simulink model "day11p2"  (R2026a)
settings: Solver=FixedStepAuto  StopTime=inf
InitFcn:
  | QueueLen = 200;
  | 
  | %{
  | fxp: udl vii hgb qmy
  | ixc: cje lra jhu
  | sgn: apv vbc
  | wua: knq
  | fnr: csd awl vvj fyx cvi xhb mvn guw wid vbp uvk krt oil izj zlh gwv
  | krt: grp cml vxt
  | hwj: laq jlg
  | rus: out
  | oag: wrc gpp
  | uos: zqg aiu gdx
  | xpu: qpb zqg gdx aiu
  | mdb: fnr mwu ozd
  | yrt: jlg ifs laq
  | eao: txi jmk xee sta knq
  | qcj: ivn mwb nrx lgx
  | wks: fyy lyd
  | xso: rqn flj fak
  | ucp: wpn mpy
  | zcf: knq sta xee jmk
  | sdr: vfy gsc wfb
  | ggn: brb ylm kdl rnk
  | tky: wcx ytk hbp xjh dne
  | kzl: sft sof utn
  | epc: uhn cqf xwv
  | srh: shh mei
  | uqe: sft
  | htw: hmf aia wsm
  | wid: qwo
  | daz: yvs
  | bdl: ipm kkp
  | xay: mpi
  | bsb: epc jpb cqs ixc cur ril ybr
  | mwb: out
  | cxr: yvs
  | ruf: jax uvl ctm
  | vtp: rbo
  | tqs: kdl pje ylm brb
  | thb: out
  | ljy: ael tqw
  | tkl: ssx yds
  | ozd: itv csd vvj fyx awl xhb mvn guw vbp hzn yft mfv izj oil uvk cui krt myo fqn gwv zlh
  | uhn: lzx dac iqf
  | zad: wvh tmc ece
  | qlf: gce sgn fni
  | kcf: dka pvw uzw
  | uat: bda mkd
  | aai: gtk gkf cuk qcj
  | mfv: cml
  | qlv: wdr sbi ihm nww jkx bud qxb
  | paz: kbq osk
  | rys: iwh
  | gdx: out
  | hco: cuk gkf
  | gte: wks fft
  | zrw: iur mei shh
  | izj: elj wrh vnz uss
  | lur: jpb zib zwl uzn epc nta cur cqs ybr tkl sle
  | ... (+518 lines)
undefined symbols (not defined in the file): DiscIntNeverNeededParam
libraries: simulink x12
(part 4 of 4)

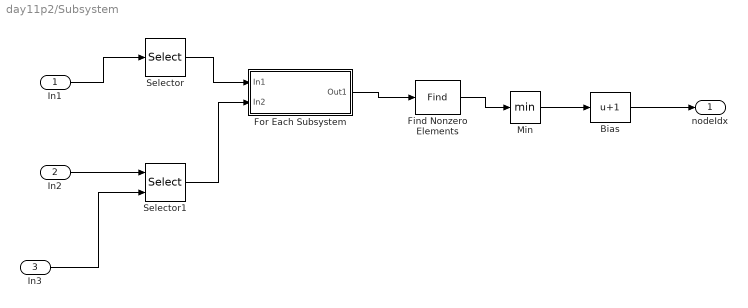
== system day11p2/Subsystem ==
  In1 : Inport
  In2 : Inport  Port=2
  In3 : Inport  Port=3
  Bias : Bias  Bias=1  SaturateOnIntegerOverflow=off
  Find Nonzero Elements : Find  NumberOfInputDimensions=3  IndexMode=Zero-based
  For Each Subsystem : Subsystem  TreatAsAtomicUnit=on
  Min : MinMax
  Selector : Selector  NumberOfDimensions=2  InputPortWidth=3  IndexOptions=Select all,Index vector (dialog)  Indices=[1 3],[1 2 3]  OutputSizes=1,1  RuntimeRangeChecks=on
  Selector1 : Selector  NumberOfDimensions=2  InputPortWidth=3  IndexOptions=Index vector (port),Index vector (dialog)  Indices=1,[1 2 3]  OutputSizes=1,1  RuntimeRangeChecks=on
  nodeIdx : Outport
  wires:
  In1/1 -> Selector/1
  In2/1 -> Selector1/1
  Selector/1 -> For Each Subsystem/1(In1)
  Selector1/1 -> For Each Subsystem/2(In2)
  For Each Subsystem/1(Out1) -> Find Nonzero Elements/1
  Find Nonzero Elements/1 -> Min/1
  Min/1 -> Bias/1
  Bias/1 -> nodeIdx/1
  In3/1 -> Selector1/2

== system day11p2/Subsystem1 ==
  In1 : Inport
  In2 : Inport  Port=2
  Assignment : Assignment  NumberOfDimensions=2  DiagnosticForDimensions=Warning  IndexOptions=Index vector (port),Index vector (dialog)  Indices=1,[1:5]  OutputSizes=1,1  RuntimeRangeChecks=on
  Bias : Bias  Bias=-1  SaturateOnIntegerOverflow=off
  Constant : Constant  Value=[0 0 0 0 0]  VectorParams1D=off
  queue : Outport
  queueLen : Outport  Port=2
  wires:
  In2/1 -> Bias/1, Assignment/3
  Bias/1 -> queueLen/1
  In1/1 -> Assignment/1
  Constant/1 -> Assignment/2
  Assignment/1 -> queue/1

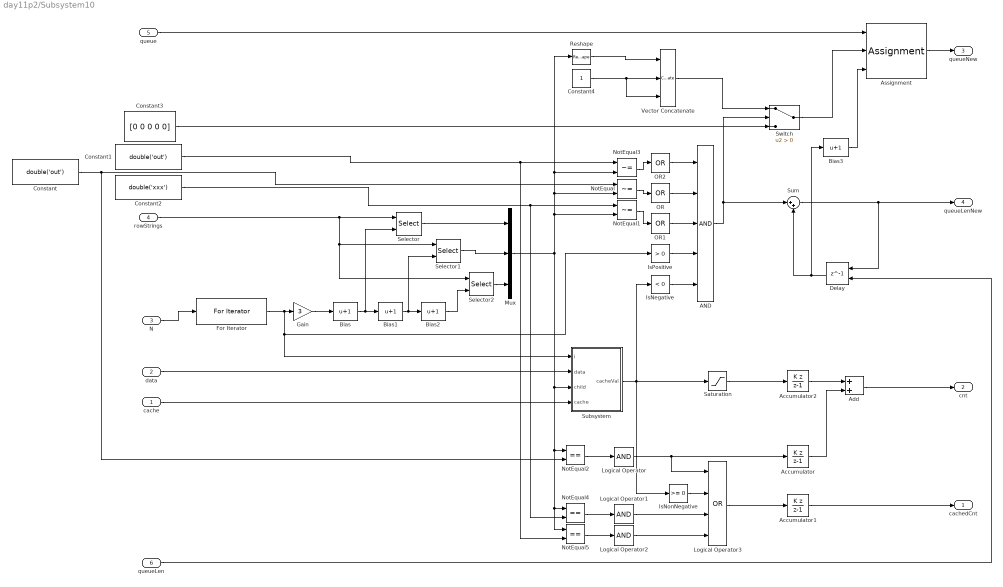
== system day11p2/Subsystem10 ==
  cache : Inport
  data : Inport  Port=2
  N : Inport  Port=3
  rowStrings : Inport  Port=4
  queue : Inport  Port=5
  queueLen : Inport  Port=6
  AND : Logic  Inputs=5  IconShape=distinctive  AllPortsSameDT=off  OutDataTypeStr=boolean
  Accumulator : DiscreteIntegrator  IntegratorMethod=Accumulation: Backward Euler  SampleTime=-1  OutDataTypeStr=double  ICPrevOutput=DiscIntNeverNeededParam  ICPrevScaledInput=DiscIntNeverNeededParam
  Accumulator1 : DiscreteIntegrator  IntegratorMethod=Accumulation: Backward Euler  SampleTime=-1  OutDataTypeStr=double  ICPrevOutput=DiscIntNeverNeededParam  ICPrevScaledInput=DiscIntNeverNeededParam
  Accumulator2 : DiscreteIntegrator  IntegratorMethod=Accumulation: Backward Euler  SampleTime=-1  OutDataTypeStr=double  ICPrevOutput=DiscIntNeverNeededParam  ICPrevScaledInput=DiscIntNeverNeededParam
  Add : Sum
  Assignment : Assignment  NumberOfDimensions=2  DiagnosticForDimensions=Warning  IndexOptions=Index vector (port),Index vector (dialog)  Indices=1,[1 2 3 4 5]  OutputSizes=1,1  RuntimeRangeChecks=on
  Bias{,1..3} (4 alike) : Bias  Bias=1  SaturateOnIntegerOverflow=off
  Constant : Constant  Value=double('out')
  Constant1 : Constant  Value=double('out')
  Constant2 : Constant  Value=double('xxx')
  Constant3 : Constant  Value=[0 0 0 0 0]  VectorParams1D=off
  Constant4 : Constant
  Delay : Delay  DelayLength=1  InitialConditionSource=Input port
      settings: InputPortMap=u0,p4
  For Iterator : ForIterator  ResetStates=reset  IterationSource=external  IndexMode=Zero-based  IterationVariableDataType=double
  Gain : Gain  Gain=3
  IsNegative : simulink/Logic and Bit Operations/Compare To Zero  relop=<  OutDataTypeStr=boolean
      settings: LibrarySourceBlock=|
      | simulink/Quick Insert/Logic and Bit
      | Operations/IsNegative
  IsNonNegative : simulink/Logic and Bit Operations/Compare To Zero  relop=>=  OutDataTypeStr=boolean
      settings: LibrarySourceBlock=|
      | simulink/Quick Insert/Logic and Bit
      | Operations/IsNonNegative
  IsPositive : simulink/Logic and Bit Operations/Compare To Zero  relop=>  OutDataTypeStr=boolean
      settings: LibrarySourceBlock=|
      | simulink/Quick Insert/Logic and Bit
      | Operations/IsPositive
  Logical Operator : Logic  Inputs=1  AllPortsSameDT=off  OutDataTypeStr=boolean
  Logical Operator1 : Logic  Inputs=1  AllPortsSameDT=off  OutDataTypeStr=boolean
  Logical Operator2 : Logic  Inputs=1  AllPortsSameDT=off  OutDataTypeStr=boolean
  Logical Operator3 : Logic  Operator=OR  Inputs=4  AllPortsSameDT=off  OutDataTypeStr=boolean
  Mux : Mux  Inputs=3
  NotEqual : RelationalOperator  Operator=~=  OutDataTypeStr=boolean  RndMeth=Simplest  InputSameDT=off
  NotEqual1 : RelationalOperator  Operator=~=  OutDataTypeStr=boolean  RndMeth=Simplest  InputSameDT=off
  NotEqual2 : RelationalOperator  Operator===  OutDataTypeStr=boolean  RndMeth=Simplest  InputSameDT=off
  NotEqual3 : RelationalOperator  Operator=~=  OutDataTypeStr=boolean  RndMeth=Simplest  InputSameDT=off
  NotEqual4 : RelationalOperator  Operator===  OutDataTypeStr=boolean  RndMeth=Simplest  InputSameDT=off
  NotEqual5 : RelationalOperator  Operator===  OutDataTypeStr=boolean  RndMeth=Simplest  InputSameDT=off
  OR : Logic  Operator=OR  Inputs=1  IconShape=distinctive  AllPortsSameDT=off  OutDataTypeStr=boolean
  OR1 : Logic  Operator=OR  Inputs=1  IconShape=distinctive  AllPortsSameDT=off  OutDataTypeStr=boolean
  OR2 : Logic  Operator=OR  Inputs=1  IconShape=distinctive  AllPortsSameDT=off  OutDataTypeStr=boolean
  Reshape : Reshape  OutputDimensionality=Row vector (2-D)
  Saturation : Saturate  UpperLimit=1e6  LowerLimit=0
  Selector : Selector  NumberOfDimensions=2  InputPortWidth=3  IndexOptions=Select all,Index vector (port)  Indices=[1 3],1  OutputSizes=1,1  RuntimeRangeChecks=on
  Selector1 : Selector  NumberOfDimensions=2  InputPortWidth=3  IndexOptions=Select all,Index vector (port)  Indices=[1 3],1  OutputSizes=1,1  RuntimeRangeChecks=on
  Selector2 : Selector  NumberOfDimensions=2  InputPortWidth=3  IndexOptions=Select all,Index vector (port)  Indices=[1 3],1  OutputSizes=1,1  RuntimeRangeChecks=on
  Subsystem : Subsystem
  Sum : Sum  Inputs=|++
  Switch : Switch  Criteria=u2 > Threshold  SaturateOnIntegerOverflow=off  InputSameDT=off
  Vector Concatenate : Concatenate  NumInputs=3
  cachedCnt : Outport
  cnt : Outport  Port=2
  queueNew : Outport  Port=3
  queueLenNew : Outport  Port=4
  wires:
  N/1 -> For Iterator/1
  Bias/1 -> Selector/2, Bias1/1
  Bias1/1 -> Selector1/2, Bias2/1
  For Iterator/1 -> Subsystem/1(i), IsPositive/1, Gain/1
  Gain/1 -> Bias/1
  rowStrings/1 -> Selector2/1, Selector1/1, Selector/1
  Bias2/1 -> Selector2/2
  Selector/1 -> Mux/1
  Selector1/1 -> Mux/2
  Selector2/1 -> Mux/3
  NotEqual/1 -> OR/1
  NotEqual1/1 -> OR1/1
  Mux/1 -> Reshape/1, NotEqual3/2, NotEqual/2, NotEqual1/2, NotEqual5/1, NotEqual4/1, NotEqual2/1, Subsystem/3(child)
  OR/1 -> AND/2
  OR1/1 -> AND/3
  IsPositive/1 -> AND/4
  Constant2/1 -> NotEqual4/2, NotEqual1/1
  AND/1 -> Sum/1, Switch/2
  Constant3/1 -> Switch/3
  Delay/1 -> Bias3/1, Sum/2
  Sum/1 -> Delay/1, queueLenNew/1
  queueLen/1 -> Delay/2
  queue/1 -> Assignment/1
  Switch/1 -> Assignment/2
  Bias3/1 -> Assignment/3
  Assignment/1 -> queueNew/1
  NotEqual2/1 -> Logical Operator/1
  Constant/1 -> NotEqual/1, NotEqual2/2
  Logical Operator/1 -> Logical Operator3/1, Accumulator/1
  Reshape/1 -> Vector Concatenate/1
  Vector Concatenate/1 -> Switch/1
  Constant4/1 -> Vector Concatenate/3, Vector Concatenate/2
  NotEqual3/1 -> OR2/1
  OR2/1 -> AND/1
  Constant1/1 -> NotEqual5/2, NotEqual3/1
  IsNegative/1 -> AND/5
  NotEqual4/1 -> Logical Operator1/1
  NotEqual5/1 -> Logical Operator2/1
  Logical Operator2/1 -> Logical Operator3/4
  Logical Operator1/1 -> Logical Operator3/3
  IsNonNegative/1 -> Logical Operator3/2
  Logical Operator3/1 -> Accumulator1/1
  Accumulator1/1 -> cachedCnt/1
  cache/1 -> Subsystem/4(cache)
  data/1 -> Subsystem/2(data)
  Subsystem/1(cacheVal) -> Saturation/1, IsNegative/1, IsNonNegative/1
  Saturation/1 -> Accumulator2/1
  Accumulator2/1 -> Add/1
  Accumulator/1 -> Add/2
  Add/1 -> cnt/1

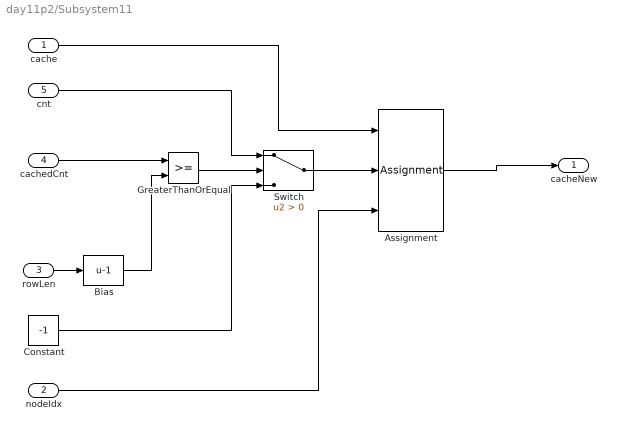
== system day11p2/Subsystem11 ==
  cache : Inport
  nodeIdx : Inport  Port=2
  rowLen : Inport  Port=3
  cachedCnt : Inport  Port=4
  cnt : Inport  Port=5
  Assignment : Assignment  DiagnosticForDimensions=Warning  IndexOptions=Index vector (port)  Indices=1  OutputSizes=1  RuntimeRangeChecks=on
  Bias : Bias  Bias=-1  SaturateOnIntegerOverflow=off
  Constant : Constant  Value=-1
  GreaterThanOrEqual : RelationalOperator  OutDataTypeStr=boolean  RndMeth=Simplest  InputSameDT=off
  Switch : Switch  Criteria=u2 > Threshold  SaturateOnIntegerOverflow=off  InputSameDT=off
  cacheNew : Outport
  wires:
  cachedCnt/1 -> GreaterThanOrEqual/1
  rowLen/1 -> Bias/1
  Bias/1 -> GreaterThanOrEqual/2
  GreaterThanOrEqual/1 -> Switch/2
  cnt/1 -> Switch/1
  Constant/1 -> Switch/3
  Switch/1 -> Assignment/2
  cache/1 -> Assignment/1
  Assignment/1 -> cacheNew/1
  nodeIdx/1 -> Assignment/3

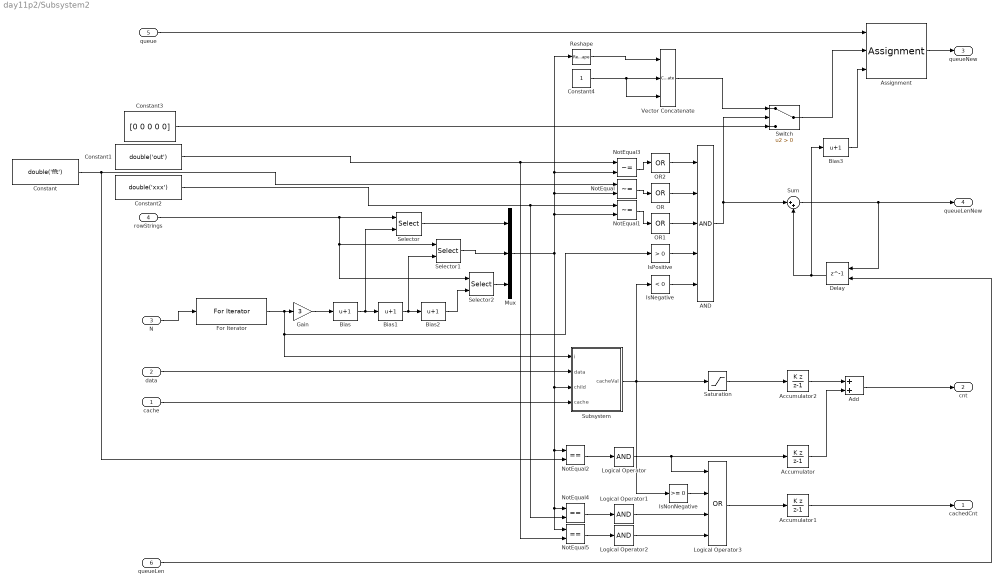
== system day11p2/Subsystem2 ==
  cache : Inport
  data : Inport  Port=2
  N : Inport  Port=3
  rowStrings : Inport  Port=4
  queue : Inport  Port=5
  queueLen : Inport  Port=6
  AND : Logic  Inputs=5  IconShape=distinctive  AllPortsSameDT=off  OutDataTypeStr=boolean
  Accumulator : DiscreteIntegrator  IntegratorMethod=Accumulation: Backward Euler  SampleTime=-1  OutDataTypeStr=double  ICPrevOutput=DiscIntNeverNeededParam  ICPrevScaledInput=DiscIntNeverNeededParam
  Accumulator1 : DiscreteIntegrator  IntegratorMethod=Accumulation: Backward Euler  SampleTime=-1  OutDataTypeStr=double  ICPrevOutput=DiscIntNeverNeededParam  ICPrevScaledInput=DiscIntNeverNeededParam
  Accumulator2 : DiscreteIntegrator  IntegratorMethod=Accumulation: Backward Euler  SampleTime=-1  OutDataTypeStr=double  ICPrevOutput=DiscIntNeverNeededParam  ICPrevScaledInput=DiscIntNeverNeededParam
  Add : Sum
  Assignment : Assignment  NumberOfDimensions=2  DiagnosticForDimensions=Warning  IndexOptions=Index vector (port),Index vector (dialog)  Indices=1,[1 2 3 4 5]  OutputSizes=1,1  RuntimeRangeChecks=on
  Bias{,1..3} (4 alike) : Bias  Bias=1  SaturateOnIntegerOverflow=off
  Constant : Constant  Value=double('fft')
  Constant1 : Constant  Value=double('out')
  Constant2 : Constant  Value=double('xxx')
  Constant3 : Constant  Value=[0 0 0 0 0]  VectorParams1D=off
  Constant4 : Constant
  Delay : Delay  DelayLength=1  InitialConditionSource=Input port
      settings: InputPortMap=u0,p4
  For Iterator : ForIterator  ResetStates=reset  IterationSource=external  IndexMode=Zero-based  IterationVariableDataType=double
  Gain : Gain  Gain=3
  IsNegative : simulink/Logic and Bit Operations/Compare To Zero  relop=<  OutDataTypeStr=boolean
      settings: LibrarySourceBlock=|
      | simulink/Quick Insert/Logic and Bit
      | Operations/IsNegative
  IsNonNegative : simulink/Logic and Bit Operations/Compare To Zero  relop=>=  OutDataTypeStr=boolean
      settings: LibrarySourceBlock=|
      | simulink/Quick Insert/Logic and Bit
      | Operations/IsNonNegative
  IsPositive : simulink/Logic and Bit Operations/Compare To Zero  relop=>  OutDataTypeStr=boolean
      settings: LibrarySourceBlock=|
      | simulink/Quick Insert/Logic and Bit
      | Operations/IsPositive
  Logical Operator : Logic  Inputs=1  AllPortsSameDT=off  OutDataTypeStr=boolean
  Logical Operator1 : Logic  Inputs=1  AllPortsSameDT=off  OutDataTypeStr=boolean
  Logical Operator2 : Logic  Inputs=1  AllPortsSameDT=off  OutDataTypeStr=boolean
  Logical Operator3 : Logic  Operator=OR  Inputs=4  AllPortsSameDT=off  OutDataTypeStr=boolean
  Mux : Mux  Inputs=3
  NotEqual : RelationalOperator  Operator=~=  OutDataTypeStr=boolean  RndMeth=Simplest  InputSameDT=off
  NotEqual1 : RelationalOperator  Operator=~=  OutDataTypeStr=boolean  RndMeth=Simplest  InputSameDT=off
  NotEqual2 : RelationalOperator  Operator===  OutDataTypeStr=boolean  RndMeth=Simplest  InputSameDT=off
  NotEqual3 : RelationalOperator  Operator=~=  OutDataTypeStr=boolean  RndMeth=Simplest  InputSameDT=off
  NotEqual4 : RelationalOperator  Operator===  OutDataTypeStr=boolean  RndMeth=Simplest  InputSameDT=off
  NotEqual5 : RelationalOperator  Operator===  OutDataTypeStr=boolean  RndMeth=Simplest  InputSameDT=off
  OR : Logic  Operator=OR  Inputs=1  IconShape=distinctive  AllPortsSameDT=off  OutDataTypeStr=boolean
  OR1 : Logic  Operator=OR  Inputs=1  IconShape=distinctive  AllPortsSameDT=off  OutDataTypeStr=boolean
  OR2 : Logic  Operator=OR  Inputs=1  IconShape=distinctive  AllPortsSameDT=off  OutDataTypeStr=boolean
  Reshape : Reshape  OutputDimensionality=Row vector (2-D)
  Saturation : Saturate  UpperLimit=1e6  LowerLimit=0
  Selector : Selector  NumberOfDimensions=2  InputPortWidth=3  IndexOptions=Select all,Index vector (port)  Indices=[1 3],1  OutputSizes=1,1  RuntimeRangeChecks=on
  Selector1 : Selector  NumberOfDimensions=2  InputPortWidth=3  IndexOptions=Select all,Index vector (port)  Indices=[1 3],1  OutputSizes=1,1  RuntimeRangeChecks=on
  Selector2 : Selector  NumberOfDimensions=2  InputPortWidth=3  IndexOptions=Select all,Index vector (port)  Indices=[1 3],1  OutputSizes=1,1  RuntimeRangeChecks=on
  Subsystem : Subsystem
  Sum : Sum  Inputs=|++
  Switch : Switch  Criteria=u2 > Threshold  SaturateOnIntegerOverflow=off  InputSameDT=off
  Vector Concatenate : Concatenate  NumInputs=3
  cachedCnt : Outport
  cnt : Outport  Port=2
  queueNew : Outport  Port=3
  queueLenNew : Outport  Port=4
  wires:
  N/1 -> For Iterator/1
  Bias/1 -> Selector/2, Bias1/1
  Bias1/1 -> Selector1/2, Bias2/1
  For Iterator/1 -> Subsystem/1(i), IsPositive/1, Gain/1
  Gain/1 -> Bias/1
  rowStrings/1 -> Selector2/1, Selector1/1, Selector/1
  Bias2/1 -> Selector2/2
  Selector/1 -> Mux/1
  Selector1/1 -> Mux/2
  Selector2/1 -> Mux/3
  NotEqual/1 -> OR/1
  NotEqual1/1 -> OR1/1
  Mux/1 -> Reshape/1, NotEqual3/2, NotEqual/2, NotEqual1/2, NotEqual5/1, NotEqual4/1, NotEqual2/1, Subsystem/3(child)
  OR/1 -> AND/2
  OR1/1 -> AND/3
  IsPositive/1 -> AND/4
  Constant2/1 -> NotEqual4/2, NotEqual1/1
  AND/1 -> Sum/1, Switch/2
  Constant3/1 -> Switch/3
  Delay/1 -> Bias3/1, Sum/2
  Sum/1 -> Delay/1, queueLenNew/1
  queueLen/1 -> Delay/2
  queue/1 -> Assignment/1
  Switch/1 -> Assignment/2
  Bias3/1 -> Assignment/3
  Assignment/1 -> queueNew/1
  NotEqual2/1 -> Logical Operator/1
  Constant/1 -> NotEqual/1, NotEqual2/2
  Logical Operator/1 -> Logical Operator3/1, Accumulator/1
  Reshape/1 -> Vector Concatenate/1
  Vector Concatenate/1 -> Switch/1
  Constant4/1 -> Vector Concatenate/3, Vector Concatenate/2
  NotEqual3/1 -> OR2/1
  OR2/1 -> AND/1
  Constant1/1 -> NotEqual5/2, NotEqual3/1
  IsNegative/1 -> AND/5
  NotEqual4/1 -> Logical Operator1/1
  NotEqual5/1 -> Logical Operator2/1
  Logical Operator2/1 -> Logical Operator3/4
  Logical Operator1/1 -> Logical Operator3/3
  IsNonNegative/1 -> Logical Operator3/2
  Logical Operator3/1 -> Accumulator1/1
  Accumulator1/1 -> cachedCnt/1
  cache/1 -> Subsystem/4(cache)
  data/1 -> Subsystem/2(data)
  Subsystem/1(cacheVal) -> Saturation/1, IsNegative/1, IsNonNegative/1
  Saturation/1 -> Accumulator2/1
  Accumulator2/1 -> Add/1
  Accumulator/1 -> Add/2
  Add/1 -> cnt/1

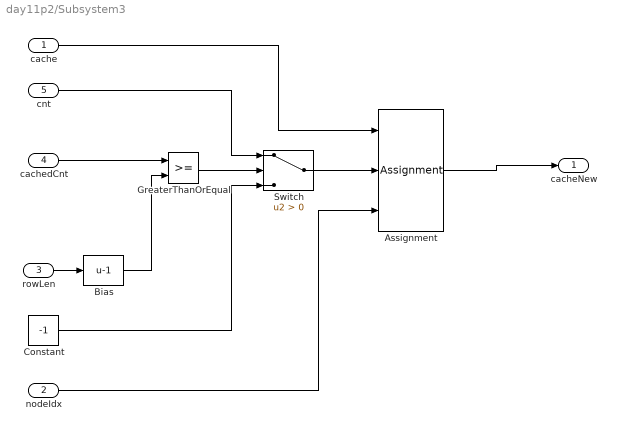
== system day11p2/Subsystem3 ==
  cache : Inport
  nodeIdx : Inport  Port=2
  rowLen : Inport  Port=3
  cachedCnt : Inport  Port=4
  cnt : Inport  Port=5
  Assignment : Assignment  DiagnosticForDimensions=Warning  IndexOptions=Index vector (port)  Indices=1  OutputSizes=1  RuntimeRangeChecks=on
  Bias : Bias  Bias=-1  SaturateOnIntegerOverflow=off
  Constant : Constant  Value=-1
  GreaterThanOrEqual : RelationalOperator  OutDataTypeStr=boolean  RndMeth=Simplest  InputSameDT=off
  Switch : Switch  Criteria=u2 > Threshold  SaturateOnIntegerOverflow=off  InputSameDT=off
  cacheNew : Outport
  wires:
  cachedCnt/1 -> GreaterThanOrEqual/1
  rowLen/1 -> Bias/1
  Bias/1 -> GreaterThanOrEqual/2
  GreaterThanOrEqual/1 -> Switch/2
  cnt/1 -> Switch/1
  Constant/1 -> Switch/3
  Switch/1 -> Assignment/2
  cache/1 -> Assignment/1
  Assignment/1 -> cacheNew/1
  nodeIdx/1 -> Assignment/3

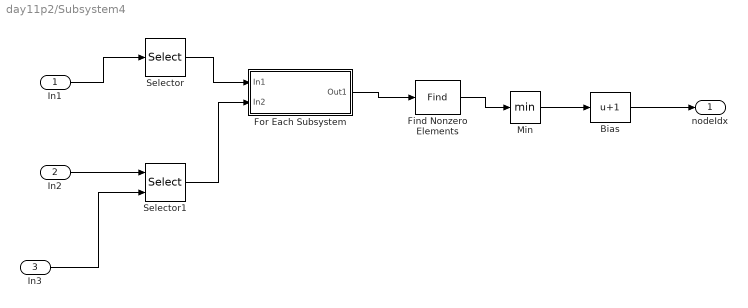
== system day11p2/Subsystem4 ==
  In1 : Inport
  In2 : Inport  Port=2
  In3 : Inport  Port=3
  Bias : Bias  Bias=1  SaturateOnIntegerOverflow=off
  Find Nonzero Elements : Find  NumberOfInputDimensions=3  IndexMode=Zero-based
  For Each Subsystem : Subsystem  TreatAsAtomicUnit=on
  Min : MinMax
  Selector : Selector  NumberOfDimensions=2  InputPortWidth=3  IndexOptions=Select all,Index vector (dialog)  Indices=[1 3],[1 2 3]  OutputSizes=1,1  RuntimeRangeChecks=on
  Selector1 : Selector  NumberOfDimensions=2  InputPortWidth=3  IndexOptions=Index vector (port),Index vector (dialog)  Indices=1,[1 2 3]  OutputSizes=1,1  RuntimeRangeChecks=on
  nodeIdx : Outport
  wires:
  In1/1 -> Selector/1
  In2/1 -> Selector1/1
  Selector/1 -> For Each Subsystem/1(In1)
  Selector1/1 -> For Each Subsystem/2(In2)
  For Each Subsystem/1(Out1) -> Find Nonzero Elements/1
  Find Nonzero Elements/1 -> Min/1
  Min/1 -> Bias/1
  Bias/1 -> nodeIdx/1
  In3/1 -> Selector1/2

== system day11p2/Subsystem5 ==
  In1 : Inport
  In2 : Inport  Port=2
  Assignment : Assignment  NumberOfDimensions=2  DiagnosticForDimensions=Warning  IndexOptions=Index vector (port),Index vector (dialog)  Indices=1,[1:5]  OutputSizes=1,1  RuntimeRangeChecks=on
  Bias : Bias  Bias=-1  SaturateOnIntegerOverflow=off
  Constant : Constant  Value=[0 0 0 0 0]  VectorParams1D=off
  queue : Outport
  queueLen : Outport  Port=2
  wires:
  In2/1 -> Bias/1, Assignment/3
  Bias/1 -> queueLen/1
  In1/1 -> Assignment/1
  Constant/1 -> Assignment/2
  Assignment/1 -> queue/1

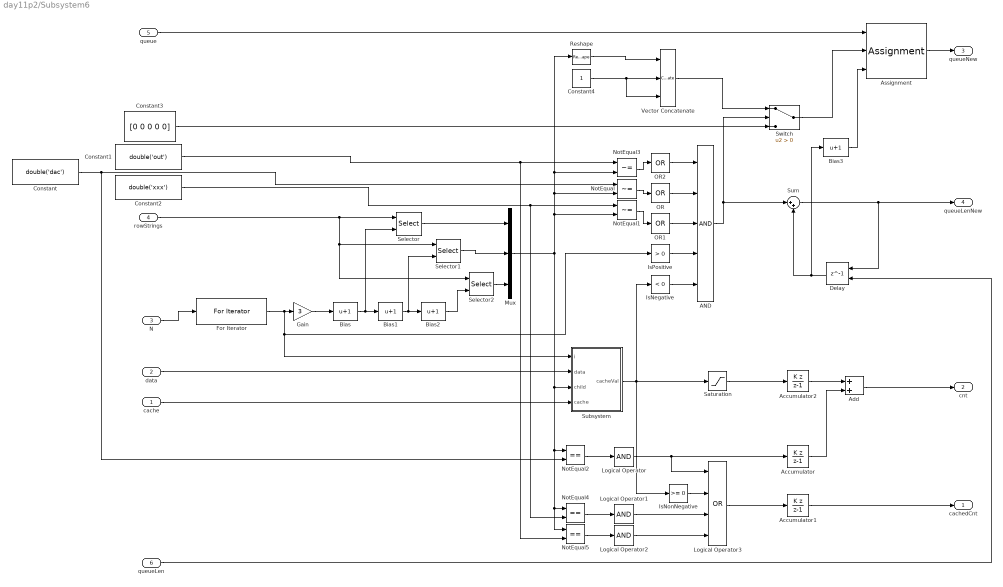
== system day11p2/Subsystem6 ==
  cache : Inport
  data : Inport  Port=2
  N : Inport  Port=3
  rowStrings : Inport  Port=4
  queue : Inport  Port=5
  queueLen : Inport  Port=6
  AND : Logic  Inputs=5  IconShape=distinctive  AllPortsSameDT=off  OutDataTypeStr=boolean
  Accumulator : DiscreteIntegrator  IntegratorMethod=Accumulation: Backward Euler  SampleTime=-1  OutDataTypeStr=double  ICPrevOutput=DiscIntNeverNeededParam  ICPrevScaledInput=DiscIntNeverNeededParam
  Accumulator1 : DiscreteIntegrator  IntegratorMethod=Accumulation: Backward Euler  SampleTime=-1  OutDataTypeStr=double  ICPrevOutput=DiscIntNeverNeededParam  ICPrevScaledInput=DiscIntNeverNeededParam
  Accumulator2 : DiscreteIntegrator  IntegratorMethod=Accumulation: Backward Euler  SampleTime=-1  OutDataTypeStr=double  ICPrevOutput=DiscIntNeverNeededParam  ICPrevScaledInput=DiscIntNeverNeededParam
  Add : Sum
  Assignment : Assignment  NumberOfDimensions=2  DiagnosticForDimensions=Warning  IndexOptions=Index vector (port),Index vector (dialog)  Indices=1,[1 2 3 4 5]  OutputSizes=1,1  RuntimeRangeChecks=on
  Bias{,1..3} (4 alike) : Bias  Bias=1  SaturateOnIntegerOverflow=off
  Constant : Constant  Value=double('dac')
  Constant1 : Constant  Value=double('out')
  Constant2 : Constant  Value=double('xxx')
  Constant3 : Constant  Value=[0 0 0 0 0]  VectorParams1D=off
  Constant4 : Constant
  Delay : Delay  DelayLength=1  InitialConditionSource=Input port
      settings: InputPortMap=u0,p4
  For Iterator : ForIterator  ResetStates=reset  IterationSource=external  IndexMode=Zero-based  IterationVariableDataType=double
  Gain : Gain  Gain=3
  IsNegative : simulink/Logic and Bit Operations/Compare To Zero  relop=<  OutDataTypeStr=boolean
      settings: LibrarySourceBlock=|
      | simulink/Quick Insert/Logic and Bit
      | Operations/IsNegative
  IsNonNegative : simulink/Logic and Bit Operations/Compare To Zero  relop=>=  OutDataTypeStr=boolean
      settings: LibrarySourceBlock=|
      | simulink/Quick Insert/Logic and Bit
      | Operations/IsNonNegative
  IsPositive : simulink/Logic and Bit Operations/Compare To Zero  relop=>  OutDataTypeStr=boolean
      settings: LibrarySourceBlock=|
      | simulink/Quick Insert/Logic and Bit
      | Operations/IsPositive
  Logical Operator : Logic  Inputs=1  AllPortsSameDT=off  OutDataTypeStr=boolean
  Logical Operator1 : Logic  Inputs=1  AllPortsSameDT=off  OutDataTypeStr=boolean
  Logical Operator2 : Logic  Inputs=1  AllPortsSameDT=off  OutDataTypeStr=boolean
  Logical Operator3 : Logic  Operator=OR  Inputs=4  AllPortsSameDT=off  OutDataTypeStr=boolean
  Mux : Mux  Inputs=3
  NotEqual : RelationalOperator  Operator=~=  OutDataTypeStr=boolean  RndMeth=Simplest  InputSameDT=off
  NotEqual1 : RelationalOperator  Operator=~=  OutDataTypeStr=boolean  RndMeth=Simplest  InputSameDT=off
  NotEqual2 : RelationalOperator  Operator===  OutDataTypeStr=boolean  RndMeth=Simplest  InputSameDT=off
  NotEqual3 : RelationalOperator  Operator=~=  OutDataTypeStr=boolean  RndMeth=Simplest  InputSameDT=off
  NotEqual4 : RelationalOperator  Operator===  OutDataTypeStr=boolean  RndMeth=Simplest  InputSameDT=off
  NotEqual5 : RelationalOperator  Operator===  OutDataTypeStr=boolean  RndMeth=Simplest  InputSameDT=off
  OR : Logic  Operator=OR  Inputs=1  IconShape=distinctive  AllPortsSameDT=off  OutDataTypeStr=boolean
  OR1 : Logic  Operator=OR  Inputs=1  IconShape=distinctive  AllPortsSameDT=off  OutDataTypeStr=boolean
  OR2 : Logic  Operator=OR  Inputs=1  IconShape=distinctive  AllPortsSameDT=off  OutDataTypeStr=boolean
  Reshape : Reshape  OutputDimensionality=Row vector (2-D)
  Saturation : Saturate  UpperLimit=1e6  LowerLimit=0
  Selector : Selector  NumberOfDimensions=2  InputPortWidth=3  IndexOptions=Select all,Index vector (port)  Indices=[1 3],1  OutputSizes=1,1  RuntimeRangeChecks=on
  Selector1 : Selector  NumberOfDimensions=2  InputPortWidth=3  IndexOptions=Select all,Index vector (port)  Indices=[1 3],1  OutputSizes=1,1  RuntimeRangeChecks=on
  Selector2 : Selector  NumberOfDimensions=2  InputPortWidth=3  IndexOptions=Select all,Index vector (port)  Indices=[1 3],1  OutputSizes=1,1  RuntimeRangeChecks=on
  Subsystem : Subsystem
  Sum : Sum  Inputs=|++
  Switch : Switch  Criteria=u2 > Threshold  SaturateOnIntegerOverflow=off  InputSameDT=off
  Vector Concatenate : Concatenate  NumInputs=3
  cachedCnt : Outport
  cnt : Outport  Port=2
  queueNew : Outport  Port=3
  queueLenNew : Outport  Port=4
  wires:
  N/1 -> For Iterator/1
  Bias/1 -> Selector/2, Bias1/1
  Bias1/1 -> Selector1/2, Bias2/1
  For Iterator/1 -> Subsystem/1(i), IsPositive/1, Gain/1
  Gain/1 -> Bias/1
  rowStrings/1 -> Selector2/1, Selector1/1, Selector/1
  Bias2/1 -> Selector2/2
  Selector/1 -> Mux/1
  Selector1/1 -> Mux/2
  Selector2/1 -> Mux/3
  NotEqual/1 -> OR/1
  NotEqual1/1 -> OR1/1
  Mux/1 -> Reshape/1, NotEqual3/2, NotEqual/2, NotEqual1/2, NotEqual5/1, NotEqual4/1, NotEqual2/1, Subsystem/3(child)
  OR/1 -> AND/2
  OR1/1 -> AND/3
  IsPositive/1 -> AND/4
  Constant2/1 -> NotEqual4/2, NotEqual1/1
  AND/1 -> Sum/1, Switch/2
  Constant3/1 -> Switch/3
  Delay/1 -> Bias3/1, Sum/2
  Sum/1 -> Delay/1, queueLenNew/1
  queueLen/1 -> Delay/2
  queue/1 -> Assignment/1
  Switch/1 -> Assignment/2
  Bias3/1 -> Assignment/3
  Assignment/1 -> queueNew/1
  NotEqual2/1 -> Logical Operator/1
  Constant/1 -> NotEqual/1, NotEqual2/2
  Logical Operator/1 -> Logical Operator3/1, Accumulator/1
  Reshape/1 -> Vector Concatenate/1
  Vector Concatenate/1 -> Switch/1
  Constant4/1 -> Vector Concatenate/3, Vector Concatenate/2
  NotEqual3/1 -> OR2/1
  OR2/1 -> AND/1
  Constant1/1 -> NotEqual5/2, NotEqual3/1
  IsNegative/1 -> AND/5
  NotEqual4/1 -> Logical Operator1/1
  NotEqual5/1 -> Logical Operator2/1
  Logical Operator2/1 -> Logical Operator3/4
  Logical Operator1/1 -> Logical Operator3/3
  IsNonNegative/1 -> Logical Operator3/2
  Logical Operator3/1 -> Accumulator1/1
  Accumulator1/1 -> cachedCnt/1
  cache/1 -> Subsystem/4(cache)
  data/1 -> Subsystem/2(data)
  Subsystem/1(cacheVal) -> Saturation/1, IsNegative/1, IsNonNegative/1
  Saturation/1 -> Accumulator2/1
  Accumulator2/1 -> Add/1
  Accumulator/1 -> Add/2
  Add/1 -> cnt/1

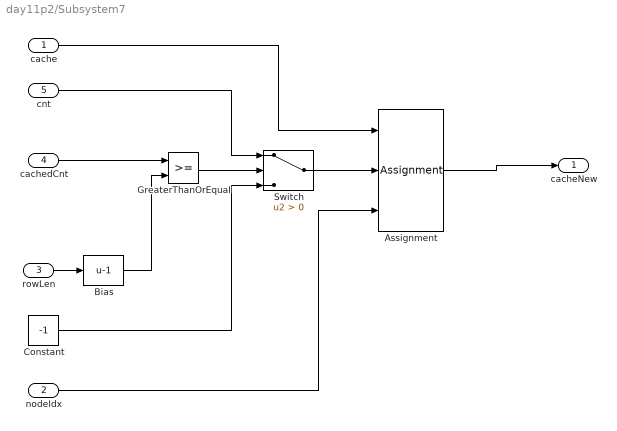
== system day11p2/Subsystem7 ==
  cache : Inport
  nodeIdx : Inport  Port=2
  rowLen : Inport  Port=3
  cachedCnt : Inport  Port=4
  cnt : Inport  Port=5
  Assignment : Assignment  DiagnosticForDimensions=Warning  IndexOptions=Index vector (port)  Indices=1  OutputSizes=1  RuntimeRangeChecks=on
  Bias : Bias  Bias=-1  SaturateOnIntegerOverflow=off
  Constant : Constant  Value=-1
  GreaterThanOrEqual : RelationalOperator  OutDataTypeStr=boolean  RndMeth=Simplest  InputSameDT=off
  Switch : Switch  Criteria=u2 > Threshold  SaturateOnIntegerOverflow=off  InputSameDT=off
  cacheNew : Outport
  wires:
  cachedCnt/1 -> GreaterThanOrEqual/1
  rowLen/1 -> Bias/1
  Bias/1 -> GreaterThanOrEqual/2
  GreaterThanOrEqual/1 -> Switch/2
  cnt/1 -> Switch/1
  Constant/1 -> Switch/3
  Switch/1 -> Assignment/2
  cache/1 -> Assignment/1
  Assignment/1 -> cacheNew/1
  nodeIdx/1 -> Assignment/3

== system day11p2/Subsystem8 ==
  In1 : Inport
  In2 : Inport  Port=2
  In3 : Inport  Port=3
  Bias : Bias  Bias=1  SaturateOnIntegerOverflow=off
  Find Nonzero Elements : Find  NumberOfInputDimensions=3  IndexMode=Zero-based
  For Each Subsystem : Subsystem  TreatAsAtomicUnit=on
  Min : MinMax
  Selector : Selector  NumberOfDimensions=2  InputPortWidth=3  IndexOptions=Select all,Index vector (dialog)  Indices=[1 3],[1 2 3]  OutputSizes=1,1  RuntimeRangeChecks=on
  Selector1 : Selector  NumberOfDimensions=2  InputPortWidth=3  IndexOptions=Index vector (port),Index vector (dialog)  Indices=1,[1 2 3]  OutputSizes=1,1  RuntimeRangeChecks=on
  nodeIdx : Outport
  wires:
  In1/1 -> Selector/1
  In2/1 -> Selector1/1
  Selector/1 -> For Each Subsystem/1(In1)
  Selector1/1 -> For Each Subsystem/2(In2)
  For Each Subsystem/1(Out1) -> Find Nonzero Elements/1
  Find Nonzero Elements/1 -> Min/1
  Min/1 -> Bias/1
  Bias/1 -> nodeIdx/1
  In3/1 -> Selector1/2

== system day11p2/Subsystem9 ==
  In1 : Inport
  In2 : Inport  Port=2
  Assignment : Assignment  NumberOfDimensions=2  DiagnosticForDimensions=Warning  IndexOptions=Index vector (port),Index vector (dialog)  Indices=1,[1:5]  OutputSizes=1,1  RuntimeRangeChecks=on
  Bias : Bias  Bias=-1  SaturateOnIntegerOverflow=off
  Constant : Constant  Value=[0 0 0 0 0]  VectorParams1D=off
  queue : Outport
  queueLen : Outport  Port=2
  wires:
  In2/1 -> Bias/1, Assignment/3
  Bias/1 -> queueLen/1
  In1/1 -> Assignment/1
  Constant/1 -> Assignment/2
  Assignment/1 -> queue/1

== system day11p2/Subsystem/For Each Subsystem ==
  In1 : Inport  Partition=on  PartitionDimension=1  PartitionWidth=1  PartitionOffset=0
  In2 : Inport  Port=2
  AND : Logic  Inputs=1  IconShape=distinctive  AllPortsSameDT=off  OutDataTypeStr=boolean
  Equal : RelationalOperator  Operator===  OutDataTypeStr=boolean  RndMeth=Simplest  InputSameDT=off
  For Each : ForEach  DisableCoverage=on
  Out1 : Outport  ConcatenationDimension=1
  wires:
  In1/1 -> Equal/1
  In2/1 -> Equal/2
  AND/1 -> Out1/1
  Equal/1 -> AND/1

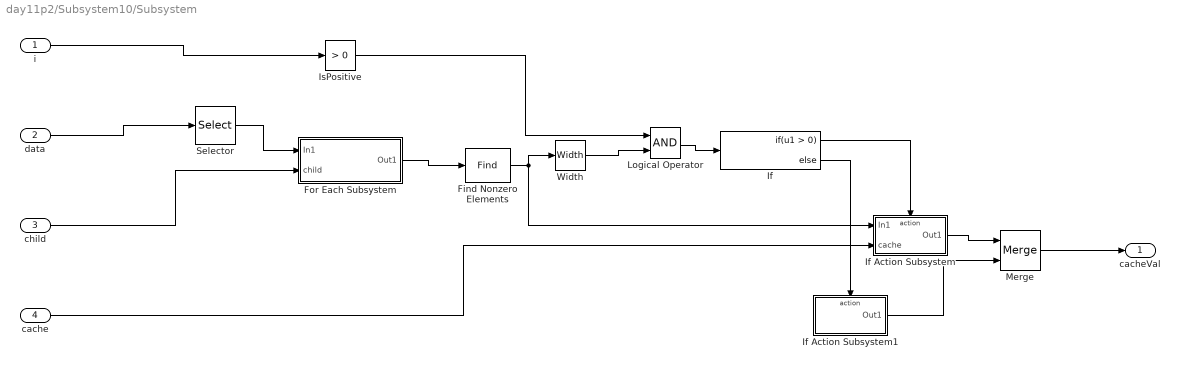
== system day11p2/Subsystem10/Subsystem ==
  i : Inport
  data : Inport  Port=2
  child : Inport  Port=3
  cache : Inport  Port=4
  Find Nonzero Elements : Find  NumberOfInputDimensions=3  IndexMode=Zero-based
  For Each Subsystem : Subsystem  TreatAsAtomicUnit=on
  If : If
  If Action Subsystem : Subsystem  TreatAsAtomicUnit=on
  If Action Subsystem1 : Subsystem  TreatAsAtomicUnit=on
  IsPositive : simulink/Logic and Bit Operations/Compare To Zero  relop=>  OutDataTypeStr=boolean
      settings: LibrarySourceBlock=|
      | simulink/Quick Insert/Logic and Bit
      | Operations/IsPositive
  Logical Operator : Logic  AllPortsSameDT=off  OutDataTypeStr=boolean
  Merge : Merge
  Selector : Selector  NumberOfDimensions=2  InputPortWidth=3  IndexOptions=Select all,Index vector (dialog)  Indices=[1 3],[1 2 3]  OutputSizes=1,1  RuntimeRangeChecks=on
  Width : Width
  cacheVal : Outport
  wires:
  data/1 -> Selector/1
  Selector/1 -> For Each Subsystem/1(In1)
  For Each Subsystem/1(Out1) -> Find Nonzero Elements/1
  child/1 -> For Each Subsystem/2(child)
  i/1 -> IsPositive/1
  Find Nonzero Elements/1 -> Width/1, If Action Subsystem/1(In1)
  IsPositive/1 -> Logical Operator/1
  Width/1 -> Logical Operator/2
  Logical Operator/1 -> If/1
  cache/1 -> If Action Subsystem/2(cache)
  If/2 -> If Action Subsystem1/Action
  If/1 -> If Action Subsystem/Action
  If Action Subsystem/1(Out1) -> Merge/1
  If Action Subsystem1/1(Out1) -> Merge/2
  Merge/1 -> cacheVal/1

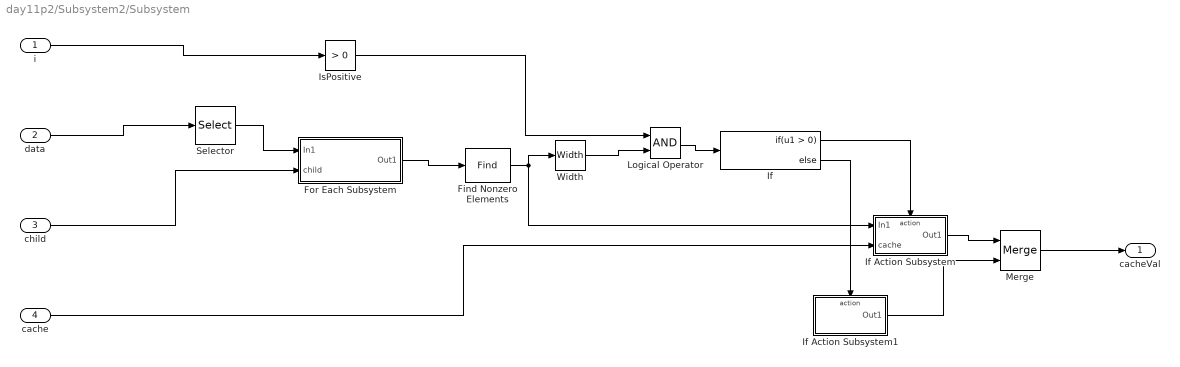
== system day11p2/Subsystem2/Subsystem ==
  i : Inport
  data : Inport  Port=2
  child : Inport  Port=3
  cache : Inport  Port=4
  Find Nonzero Elements : Find  NumberOfInputDimensions=3  IndexMode=Zero-based
  For Each Subsystem : Subsystem  TreatAsAtomicUnit=on
  If : If
  If Action Subsystem : Subsystem  TreatAsAtomicUnit=on
  If Action Subsystem1 : Subsystem  TreatAsAtomicUnit=on
  IsPositive : simulink/Logic and Bit Operations/Compare To Zero  relop=>  OutDataTypeStr=boolean
      settings: LibrarySourceBlock=|
      | simulink/Quick Insert/Logic and Bit
      | Operations/IsPositive
  Logical Operator : Logic  AllPortsSameDT=off  OutDataTypeStr=boolean
  Merge : Merge
  Selector : Selector  NumberOfDimensions=2  InputPortWidth=3  IndexOptions=Select all,Index vector (dialog)  Indices=[1 3],[1 2 3]  OutputSizes=1,1  RuntimeRangeChecks=on
  Width : Width
  cacheVal : Outport
  wires:
  data/1 -> Selector/1
  Selector/1 -> For Each Subsystem/1(In1)
  For Each Subsystem/1(Out1) -> Find Nonzero Elements/1
  child/1 -> For Each Subsystem/2(child)
  i/1 -> IsPositive/1
  Find Nonzero Elements/1 -> Width/1, If Action Subsystem/1(In1)
  IsPositive/1 -> Logical Operator/1
  Width/1 -> Logical Operator/2
  Logical Operator/1 -> If/1
  cache/1 -> If Action Subsystem/2(cache)
  If/2 -> If Action Subsystem1/Action
  If/1 -> If Action Subsystem/Action
  If Action Subsystem/1(Out1) -> Merge/1
  If Action Subsystem1/1(Out1) -> Merge/2
  Merge/1 -> cacheVal/1

== system day11p2/Subsystem4/For Each Subsystem ==
  In1 : Inport  Partition=on  PartitionDimension=1  PartitionWidth=1  PartitionOffset=0
  In2 : Inport  Port=2
  AND : Logic  Inputs=1  IconShape=distinctive  AllPortsSameDT=off  OutDataTypeStr=boolean
  Equal : RelationalOperator  Operator===  OutDataTypeStr=boolean  RndMeth=Simplest  InputSameDT=off
  For Each : ForEach  DisableCoverage=on
  Out1 : Outport  ConcatenationDimension=1
  wires:
  In1/1 -> Equal/1
  In2/1 -> Equal/2
  AND/1 -> Out1/1
  Equal/1 -> AND/1

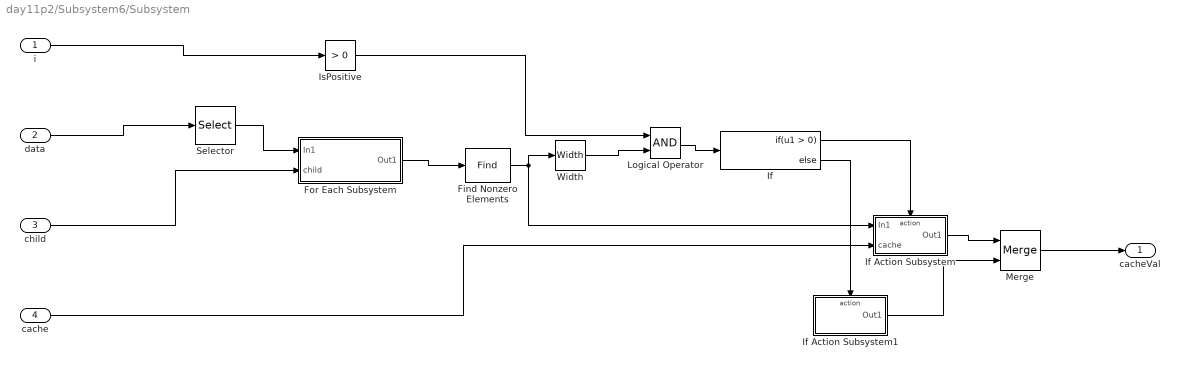
== system day11p2/Subsystem6/Subsystem ==
  i : Inport
  data : Inport  Port=2
  child : Inport  Port=3
  cache : Inport  Port=4
  Find Nonzero Elements : Find  NumberOfInputDimensions=3  IndexMode=Zero-based
  For Each Subsystem : Subsystem  TreatAsAtomicUnit=on
  If : If
  If Action Subsystem : Subsystem  TreatAsAtomicUnit=on
  If Action Subsystem1 : Subsystem  TreatAsAtomicUnit=on
  IsPositive : simulink/Logic and Bit Operations/Compare To Zero  relop=>  OutDataTypeStr=boolean
      settings: LibrarySourceBlock=|
      | simulink/Quick Insert/Logic and Bit
      | Operations/IsPositive
  Logical Operator : Logic  AllPortsSameDT=off  OutDataTypeStr=boolean
  Merge : Merge
  Selector : Selector  NumberOfDimensions=2  InputPortWidth=3  IndexOptions=Select all,Index vector (dialog)  Indices=[1 3],[1 2 3]  OutputSizes=1,1  RuntimeRangeChecks=on
  Width : Width
  cacheVal : Outport
  wires:
  data/1 -> Selector/1
  Selector/1 -> For Each Subsystem/1(In1)
  For Each Subsystem/1(Out1) -> Find Nonzero Elements/1
  child/1 -> For Each Subsystem/2(child)
  i/1 -> IsPositive/1
  Find Nonzero Elements/1 -> Width/1, If Action Subsystem/1(In1)
  IsPositive/1 -> Logical Operator/1
  Width/1 -> Logical Operator/2
  Logical Operator/1 -> If/1
  cache/1 -> If Action Subsystem/2(cache)
  If/2 -> If Action Subsystem1/Action
  If/1 -> If Action Subsystem/Action
  If Action Subsystem/1(Out1) -> Merge/1
  If Action Subsystem1/1(Out1) -> Merge/2
  Merge/1 -> cacheVal/1

== system day11p2/Subsystem8/For Each Subsystem ==
  In1 : Inport  Partition=on  PartitionDimension=1  PartitionWidth=1  PartitionOffset=0
  In2 : Inport  Port=2
  AND : Logic  Inputs=1  IconShape=distinctive  AllPortsSameDT=off  OutDataTypeStr=boolean
  Equal : RelationalOperator  Operator===  OutDataTypeStr=boolean  RndMeth=Simplest  InputSameDT=off
  For Each : ForEach  DisableCoverage=on
  Out1 : Outport  ConcatenationDimension=1
  wires:
  In1/1 -> Equal/1
  In2/1 -> Equal/2
  AND/1 -> Out1/1
  Equal/1 -> AND/1

== system day11p2/Subsystem10/Subsystem/For Each Subsystem ==
  In1 : Inport  Partition=on  PartitionDimension=1  PartitionWidth=1  PartitionOffset=0
  child : Inport  Port=2
  AND : Logic  Inputs=1  IconShape=distinctive  AllPortsSameDT=off  OutDataTypeStr=boolean
  Equal : RelationalOperator  Operator===  OutDataTypeStr=boolean  RndMeth=Simplest  InputSameDT=off
  For Each : ForEach  DisableCoverage=on
  Out1 : Outport  ConcatenationDimension=1
  wires:
  In1/1 -> Equal/1
  child/1 -> Equal/2
  AND/1 -> Out1/1
  Equal/1 -> AND/1

== system day11p2/Subsystem10/Subsystem/If Action Subsystem ==
  In1 : Inport
  cache : Inport  Port=2
  Action Port : ActionPort  ActionPortLabel=if(u1 > 0)
  Bias : Bias  Bias=1  SaturateOnIntegerOverflow=off
  Cast To Double : DataTypeConversion  OutDataTypeStr=double  SaturateOnIntegerOverflow=off  RndMeth=Floor
  Min1 : MinMax
  Selector : Selector  NumberOfDimensions=2  InputPortWidth=3  IndexOptions=Index vector (port),Select all  Indices=[1 3],1  OutputSizes=1,1  RuntimeRangeChecks=on
  Out1 : Outport
  wires:
  In1/1 -> Min1/1
  Min1/1 -> Cast To Double/1
  Cast To Double/1 -> Bias/1
  cache/1 -> Selector/1
  Bias/1 -> Selector/2
  Selector/1 -> Out1/1

== system day11p2/Subsystem10/Subsystem/If Action Subsystem1 ==
  Action Port : ActionPort  ActionPortLabel=else
  Constant : Constant  Value=-1
  Out1 : Outport
  wires:
  Constant/1 -> Out1/1

== system day11p2/Subsystem2/Subsystem/For Each Subsystem ==
  In1 : Inport  Partition=on  PartitionDimension=1  PartitionWidth=1  PartitionOffset=0
  child : Inport  Port=2
  AND : Logic  Inputs=1  IconShape=distinctive  AllPortsSameDT=off  OutDataTypeStr=boolean
  Equal : RelationalOperator  Operator===  OutDataTypeStr=boolean  RndMeth=Simplest  InputSameDT=off
  For Each : ForEach  DisableCoverage=on
  Out1 : Outport  ConcatenationDimension=1
  wires:
  In1/1 -> Equal/1
  child/1 -> Equal/2
  AND/1 -> Out1/1
  Equal/1 -> AND/1

== system day11p2/Subsystem2/Subsystem/If Action Subsystem ==
  In1 : Inport
  cache : Inport  Port=2
  Action Port : ActionPort  ActionPortLabel=if(u1 > 0)
  Bias : Bias  Bias=1  SaturateOnIntegerOverflow=off
  Cast To Double : DataTypeConversion  OutDataTypeStr=double  SaturateOnIntegerOverflow=off  RndMeth=Floor
  Min1 : MinMax
  Selector : Selector  NumberOfDimensions=2  InputPortWidth=3  IndexOptions=Index vector (port),Select all  Indices=[1 3],1  OutputSizes=1,1  RuntimeRangeChecks=on
  Out1 : Outport
  wires:
  In1/1 -> Min1/1
  Min1/1 -> Cast To Double/1
  Cast To Double/1 -> Bias/1
  cache/1 -> Selector/1
  Bias/1 -> Selector/2
  Selector/1 -> Out1/1

== system day11p2/Subsystem2/Subsystem/If Action Subsystem1 ==
  Action Port : ActionPort  ActionPortLabel=else
  Constant : Constant  Value=-1
  Out1 : Outport
  wires:
  Constant/1 -> Out1/1

== system day11p2/Subsystem6/Subsystem/For Each Subsystem ==
  In1 : Inport  Partition=on  PartitionDimension=1  PartitionWidth=1  PartitionOffset=0
  child : Inport  Port=2
  AND : Logic  Inputs=1  IconShape=distinctive  AllPortsSameDT=off  OutDataTypeStr=boolean
  Equal : RelationalOperator  Operator===  OutDataTypeStr=boolean  RndMeth=Simplest  InputSameDT=off
  For Each : ForEach  DisableCoverage=on
  Out1 : Outport  ConcatenationDimension=1
  wires:
  In1/1 -> Equal/1
  child/1 -> Equal/2
  AND/1 -> Out1/1
  Equal/1 -> AND/1

== system day11p2/Subsystem6/Subsystem/If Action Subsystem ==
  In1 : Inport
  cache : Inport  Port=2
  Action Port : ActionPort  ActionPortLabel=if(u1 > 0)
  Bias : Bias  Bias=1  SaturateOnIntegerOverflow=off
  Cast To Double : DataTypeConversion  OutDataTypeStr=double  SaturateOnIntegerOverflow=off  RndMeth=Floor
  Min1 : MinMax
  Selector : Selector  NumberOfDimensions=2  InputPortWidth=3  IndexOptions=Index vector (port),Select all  Indices=[1 3],1  OutputSizes=1,1  RuntimeRangeChecks=on
  Out1 : Outport
  wires:
  In1/1 -> Min1/1
  Min1/1 -> Cast To Double/1
  Cast To Double/1 -> Bias/1
  cache/1 -> Selector/1
  Bias/1 -> Selector/2
  Selector/1 -> Out1/1

== system day11p2/Subsystem6/Subsystem/If Action Subsystem1 ==
  Action Port : ActionPort  ActionPortLabel=else
  Constant : Constant  Value=-1
  Out1 : Outport
  wires:
  Constant/1 -> Out1/1
